simulink model "room207_gazebo"  (R2026b)
settings: Solver=ode15s  StopTime=inf  RelTol=1e-6  AbsTol=1e-8
PreLoadFcn:
  | if exist('room207_setup', 'file'), room207_setup(); end
StartFcn:
  | room207.viewer('start', bdroot, {'Simulink LIMO (twin)', 'Gazebo LIMO (/odom)'});
StopFcn:
  | room207.viewer('stop');
undefined symbols (not defined in the file or in its folder): angular, linear
libraries: ros2lib x3, limo_lib x1
settings Model: Creator=jkreiss  LastModifiedBy=jkreiss
settings DataIOCC: SaveOutput=off  SaveTime=off

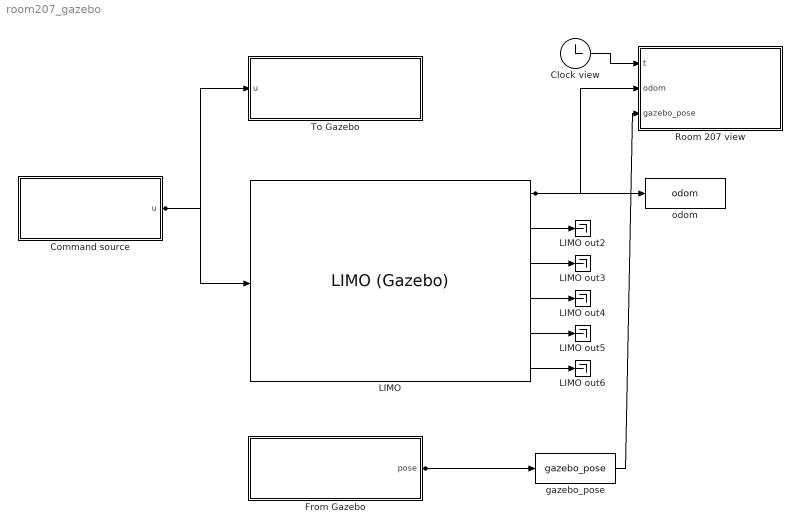
== system room207_gazebo ==
  Clock view : Clock
  Command source : Subsystem
  From Gazebo : Subsystem
  LIMO : limo_lib/LIMO (Gazebo)  input_mode=Steering angle: [v; gamma]  pose_mode=Room 207 spawn  custom_pose=[0 0 0]  mu=1  v_eps=1e-3
      settings: SourceProductName=LIMO (ENSEM)
  LIMO out{2..6} (5 alike) : Terminator
  Room 207 view : MATLAB Function  TreatAsAtomicUnit=on  SystemSampleTime=0.05
  To Gazebo : Subsystem
  gazebo_pose : ToWorkspace  VariableName=gazebo_pose  SaveFormat=Timeseries  SampleTime=-1
  odom : ToWorkspace  VariableName=odom  SaveFormat=Timeseries  SampleTime=-1
  wires:
  Command source/1(u) -> LIMO/1, To Gazebo/1(u)
  Clock view/1 -> Room 207 view/1(t)
  LIMO/1 -> Room 207 view/2(odom), odom/1
  From Gazebo/1(pose) -> Room 207 view/3(gazebo_pose), gazebo_pose/1
  LIMO/2 -> LIMO out2/1
  LIMO/3 -> LIMO out3/1
  LIMO/4 -> LIMO out4/1
  LIMO/5 -> LIMO out5/1
  LIMO/6 -> LIMO out6/1

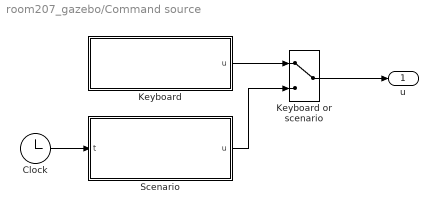
== system room207_gazebo/Command source ==
  Clock : Clock
  Keyboard : MATLAB Function  TreatAsAtomicUnit=on  SystemSampleTime=0.05
  Keyboard or scenario : ManualSwitch
  Scenario : MATLAB Function  TreatAsAtomicUnit=on
  u : Outport
  wires:
  Scenario/1(u) -> Keyboard or scenario/2
  Clock/1 -> Scenario/1(t)
  Keyboard/1(u) -> Keyboard or scenario/1
  Keyboard or scenario/1 -> u/1

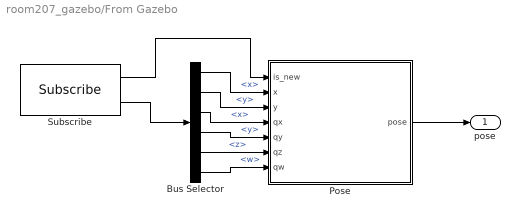
== system room207_gazebo/From Gazebo ==
  Bus Selector : BusSelector  OutputSignals=pose.pose.position.x,pose.pose.position.y,pose.pose.orientation.x,pose.pose.orientation.y,pose.pose.orientation.z,pose.pose.orientation.w
  Pose : MATLAB Function  TreatAsAtomicUnit=on
  Subscribe : ros2lib/Subscribe  topicSource=Specify your own  topic=/odom  messageType=nav_msgs/Odometry  SubscriberMode=At sample time  sampleTime=0.05  CallbackGroupType=Default  CallbackGroupName=callback_group_1  QOSHistory=Keep last  QOSDepth=10  QOSReliability=Reliable  QOSDurability=Volatile  QOSDeadline=Inf  QOSLifespan=Inf  QOSLiveliness=Automatic  QOSLeaseDuration=Inf  QOSAvoidROSNamespaceConventions=off
  pose : Outport
  wires:
  Subscribe/1 -> Pose/1(is_new)
  Subscribe/2 -> Bus Selector/1
  Bus Selector/1 -> Pose/2(x)  "<x>"
  Bus Selector/2 -> Pose/3(y)  "<y>"
  Bus Selector/3 -> Pose/4(qx)  "<x>"
  Bus Selector/4 -> Pose/5(qy)  "<y>"
  Bus Selector/5 -> Pose/6(qz)  "<z>"
  Bus Selector/6 -> Pose/7(qw)  "<w>"
  Pose/1(pose) -> pose/1

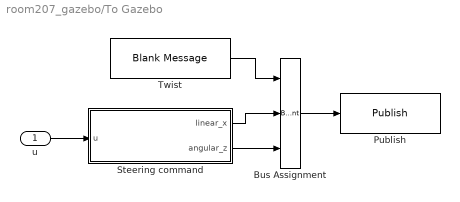
== system room207_gazebo/To Gazebo ==
  u : Inport
  Bus Assignment : BusAssignment  AssignedSignals=linear.x,angular.z
  Publish : ros2lib/Publish  topicSource=Specify your own  topic=/cmd_vel_gazebo  messageType=geometry_msgs/Twist  QOSHistory=Keep last  QOSDepth=10  QOSReliability=Reliable  QOSDurability=Volatile  QOSDeadline=Inf  QOSLifespan=Inf  QOSLiveliness=Automatic  QOSLeaseDuration=Inf  QOSAvoidROSNamespaceConventions=off
  Steering command : MATLAB Function  TreatAsAtomicUnit=on  SystemSampleTime=0.05
  Twist : ros2lib/Blank Message  messageClass=Message  entityType=geometry_msgs/Twist  messageType=geometry_msgs/Twist  SampleTime=0.05
  wires:
  Twist/1 -> Bus Assignment/1
  u/1 -> Steering command/1(u)
  Steering command/2(angular_z) -> Bus Assignment/3
  Steering command/1(linear_x) -> Bus Assignment/2
  Bus Assignment/1 -> Publish/1

== matlab function room207_gazebo/Command source/Scenario ==
  data: t input; u output
function u = scenario(t)
%SCENARIO Speed and steering angle as a function of time.
%   u = [v (m/s); gamma (rad)], gamma > 0 to the left
%
%   From the Room 207 spawn: leave the parking bay, turn left into the
%   car park, stop, then reverse along the same arc back into the bay.

v = 0;
gamma = 0;

if t >= 1 && t < 7.3
    v = 0.3;
elseif t >= 8 && t < 14.3
    v = -0.3;
end

if (t >= 4.3 && t < 7.3) || (t >= 8 && t < 11)
    gamma = 0.35;
end

u = [v; gamma];

== matlab function room207_gazebo/Command source/Keyboard ==
  data: u output
function u = keyboard_command()
%KEYBOARD_COMMAND [v; gamma] from the keyboard (room207.viewer).
%   Z/S: forward/backward, Q/D: left/right, Space: stop, Esc: end.

coder.extrinsic('room207.viewer');

u = zeros(2, 1);
u = room207.viewer('command');

== matlab function room207_gazebo/To Gazebo/Steering command ==
  data: u input; linear_x output; angular_z output
function [linear_x, angular_z] = steering(u)
%STEERING [v; gamma] -> /cmd_vel_gazebo (limo.gazebo_steering_command).

cmd = limo.gazebo_steering_command(u(1), u(2));
linear_x = cmd(1);
angular_z = cmd(2);

== matlab function room207_gazebo/From Gazebo/Pose ==
  data: is_new input; pose output; x input; y input; qx input; qy input; qz input; qw input
function pose = odom_pose(is_new, x, y, qx, qy, qz, qw)
%ODOM_POSE Last [X; Y; psi] received on /odom (NaN before the first).

persistent last

if isempty(last)
    last = nan(3, 1);
end

if is_new
    psi = atan2(2*(qw*qz + qx*qy), 1 - 2*(qy^2 + qz^2));
    last = [x; y; psi];
end

pose = last;

== matlab function room207_gazebo/Room 207 view ==
  data: t input; odom input; gazebo_pose input
function view(t, odom, gazebo_pose)
%VIEW Draw the Simulink twin and the Gazebo LIMO (room207.viewer).

coder.extrinsic('room207.viewer');

room207.viewer('draw', t, [odom(1:3), gazebo_pose]);
